simulink model "ErrorAnalyzer"  (R2025b)
settings: Solver=VariableStepAuto  StartTime=0.0  StopTime=10.0  RelTol=1e-3
settings Model: Creator=Ishwar  LastModifiedBy=Ishwar

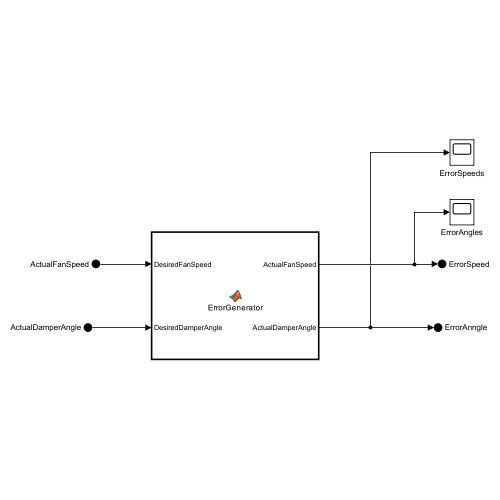
[thumbnail: Simulink's stored preview of the top-level diagram]
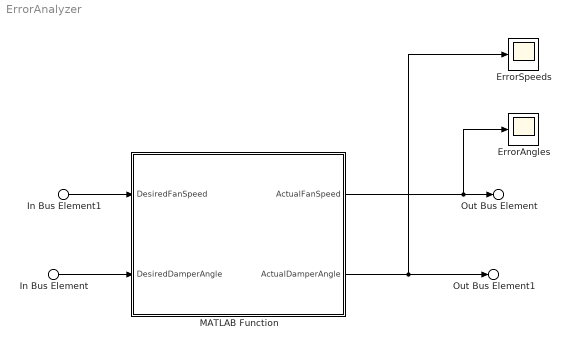
== system ErrorAnalyzer ==
  In Bus Element : Inport  PortName=ActualDamperAngle
  In Bus Element1 : Inport  Port=2  PortName=ActualFanSpeed
  ErrorAngles : Scope
      settings: ActiveDisplayYMinimum=40.693333333333335  ActiveDisplayYMaximum=53.193333333333335
  ErrorSpeeds : Scope
      settings: ActiveDisplayYMinimum=33.219846014492745  ActiveDisplayYMaximum=41.094846014492745
  MATLAB Function : MATLAB Function  TreatAsAtomicUnit=on
  Out Bus Element : Outport  PortName=ErrorFanSpeed
  Out Bus Element1 : Outport  Port=2  PortName=ErrorDamperAngle
  wires:
  In Bus Element/1 -> MATLAB Function/2(DesiredDamperAngle)
  In Bus Element1/1 -> MATLAB Function/1(DesiredFanSpeed)
  MATLAB Function/2(ActualDamperAngle) -> ErrorSpeeds/1, Out Bus Element1/1
  MATLAB Function/1(ActualFanSpeed) -> ErrorAngles/1, Out Bus Element/1

== matlab function ErrorAnalyzer/MATLAB Function ==
  data: DesiredFanSpeed input; ActualFanSpeed output; DesiredDamperAngle input; ActualDamperAngle output
function [ActualFanSpeed, ActualDamperAngle] = ErrorGenerator(DesiredFanSpeed, DesiredDamperAngle)
%#codegen

% Inject random deviation
fanNoise    = randi([-5, 4]);   % ±5% deviation
damperNoise = randi([-3, 6]);   % ±3° deviation

% Simulate actuator mismatch
ActualFanSpeed   = DesiredFanSpeed + fanNoise;
ActualDamperAngle = DesiredDamperAngle + damperNoise;

% Clamp values to safe ranges
ActualFanSpeed   = max(0, min(100, ActualFanSpeed));
ActualDamperAngle = max(0, min(90, ActualDamperAngle));
